simulink model "reglet_damping_variant_g"  (R2024b)
settings: Solver=VariableStepAuto  StartTime=0.0  StopTime=6  MaxStep=1e-3  RelTol=1e-3  AbsTol=1e-3  EnableMultiTasking=on
libraries: fl_lib x18, nesl_utility x6, simulink x1
CloseFcn:
  | try,close(h1_PermanentMagnetDCMotor),end
  | clear h1_PermanentMagnetDCMotor
  | 
  | clear simlog_PermanentMagnetDCMotor
Description:
  | Permanent Magnet DC Motor
settings Model: Creator=The MathWorks, Inc.  LastModifiedBy=thurard609
settings SolverCC: AutoScaleAbsTol=off  AlgebraicLoopSolver=TrustRegion
settings DataIOCC: LimitDataPoints=on  SaveFormat=Array  ReturnWorkspaceOutputs=off
settings OptimizationCC: ReuseModelBlockBuffer=off  LifeSpan=inf
settings DebuggingCC: SolverPrmCheckMsg=warning  UnconnectedInputMsg=warning  UnconnectedOutputMsg=warning  UnconnectedLineMsg=warning  AllowSymbolicDim=off  PregeneratedLibrarySubsystemCodeDiagnostic=none  SFUnexpectedBacktrackingDiag=warning  SFNoUnconditionalDefaultTransitionDiag=warning  SFExecutionAtInitializationDiag=none  ArithmeticOperatorsInVariantConditions=warning
settings HardwareCC: ProdBitPerPointer=32  ProdBitPerSizeT=32  ProdBitPerPtrDiffT=32  ProdLargestAtomicFloat=None  ProdIntDivRoundTo=Undefined  ProdEndianess=Unspecified  ProdWordSize=32  ProdHWDeviceType=32-bit Generic
settings ModelReferenceCC: EnableRefExpFcnMdlSchedulingChecks=on  PropagateSignalLabelsOutOfModel=off
settings SFSimCC: SimUseLocalCustomCode=off  CustomCodeUndefinedFunction=UseInterfaceOnly
settings RTWCC: RTWUseLocalCustomCode=off  GPUComputeCapability=3.5  DLArmComputeVersion=19.05
settings CodeAppCC: StateflowObjectComments=on
settings GRTTargetCC: TargetLangStandard=C89/C90 (ANSI)
settings ConfigComp: CovMetricSettings=dw  CovSaveCumulativeToWorkspaceVar=on  CovSaveSingleToWorkspaceVar=on  CovExternalEMLEnable=off  CovSFcnEnable=off
settings SimscapeCC: SimscapeLogType=all  SimscapeLogSimulationStatistics=on  SimscapeLogName=simlog_PermanentMagnetDCMotor  SimscapeLogDataHistory=10000

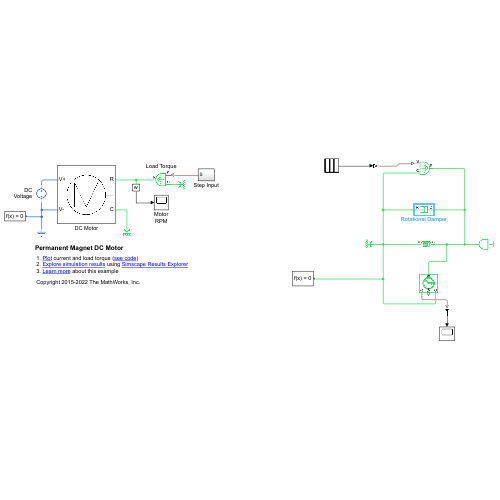
[thumbnail: Simulink's stored preview of the top-level diagram]
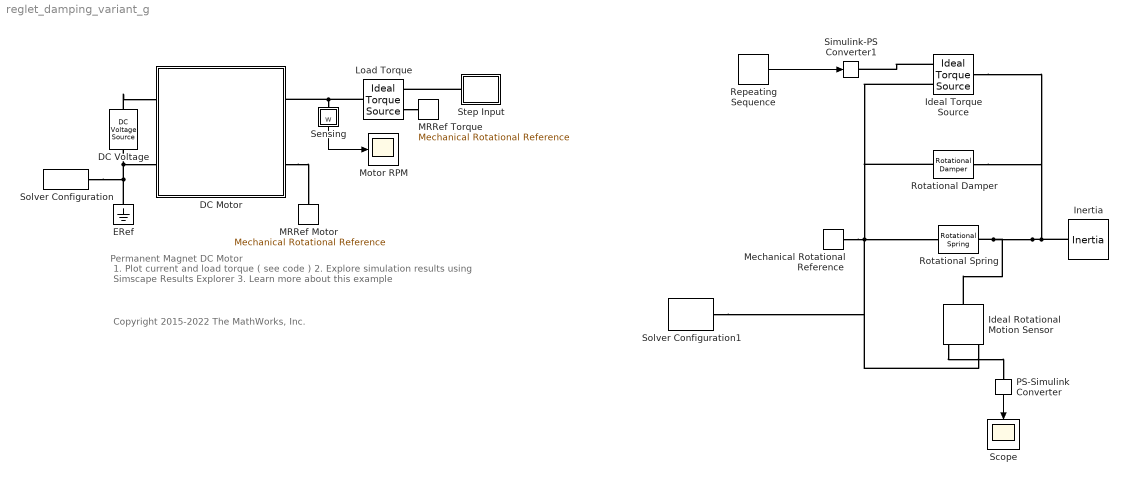
== system reglet_damping_variant_g ==
  note: 1. Plot current and load torque ( see code )
      | 2. Explore simulation results using Simscape Results Explorer
      | 3. Learn more about this example
  note: Permanent Magnet DC Motor
  note: Copyright 2015-2022 The MathWorks, Inc.
  DC Voltage : fl_lib/Electrical/Electrical Sources/DC Voltage Source  v0=1.5 V
  DC Motor : Subsystem  Tag=PublishSubsystem
      mask Display:
      | % Circle, in/out, and 'M'
      | image('PermanentMagnetDCMotorMaskIcon.png');
      | 
      | % % Circle
      | % plot(sin(0:0.1:2.2*pi)*0.9,cos(0:0.1:2.2*pi)*0.9);
      | %
      | % % In/out
      | % plot([-1.3 -0.9],[0 0]);
      | % plot([1.3 0.9],[0 0]);
      | %
      | % % 'M'
      | % plot([0.5 0.5],[-0.5 0.5]);
      | % plot([-0.5 -0.5],[-0.5 0.5]);
      | % plot([0.5 0],[0.5 -0.5]);
      | % plot([-0.5 0],[0.5 -0.5]);
      | 
      | % Plot points to set plot range
      | color('white');plot(1.5,1.5);plot(-1.5,-1.5)
      | color('black');
      | 
      | port_label('RConn',1,'R');
      | port_label('RConn',2,'C');
      | port_label('LConn',1,'V+');
      | port_label('LConn',2,'V-');
  ERef : fl_lib/Electrical/Electrical Elements/Electrical Reference
  Ideal Rotational Motion Sensor : fl_lib/Mechanical/Mechanical Sensors/Ideal Rotational Motion Sensor  reference=foundation.enum.MeasurementReference.difference  acceleration_port=false  velocity_port=true  position_port=true  wrap_angle=false  offset=0 rad
  Ideal Torque Source : fl_lib/Mechanical/Mechanical Sources/Ideal Torque Source
  Inertia : fl_lib/Mechanical/Rotational Elements/Inertia  inertia=9e-4 kg*m^2  num_ports=foundation.enum.numPorts2.one  w_specify=off  w_priority=High  w=0 rad/s  w_nominal_specify=off  w_nominal_value=1  w_nominal_unit=rad/s  t_specify=off  t_priority=None  t=0 N*m  t_nominal_specify=off  t_nominal_value=1  t_nominal_unit=N*m
  Load Torque : fl_lib/Mechanical/Mechanical Sources/Ideal Torque Source
  MRRef Motor : fl_lib/Mechanical/Rotational Elements/Mechanical Rotational Reference
  MRRef Torque : fl_lib/Mechanical/Rotational Elements/Mechanical Rotational Reference
  Mechanical Rotational Reference : fl_lib/Mechanical/Rotational Elements/Mechanical Rotational Reference
  Motor RPM : Scope
  PS-Simulink Converter : nesl_utility/PS-Simulink Converter  PhysicalDomain=network_engine_domain  SubClassName=ps_output  LeftPortType=input  RightPortType=output  PseudoPeriodic=off  Frequencies=[]  VectorFormat=inherit  Unit=rad  AffineConversion=off
  Repeating Sequence : simulink/Sources/Repeating Sequence  rep_seq_t=[0 0.01 0.02 0.03 6]  rep_seq_y=[0 0.05 0.05 0 0]
  Rotational Damper : fl_lib/Mechanical/Rotational Elements/Rotational Damper  D=1.661e-3 N*m*s/rad  w_specify=off  w_priority=None  w=0 rad/s  w_nominal_specify=off  w_nominal_value=1  w_nominal_unit=rad/s  t_specify=off  t_priority=None  t=0 N*m  t_nominal_specify=off  t_nominal_value=1  t_nominal_unit=N*m
  Rotational Spring : fl_lib/Mechanical/Rotational Elements/Rotational Spring  spr_rate=0.4476 N*m/rad  w_specify=off  w_priority=None  w=0 rad/s  w_nominal_specify=off  w_nominal_value=1  w_nominal_unit=rad/s  t_specify=off  t_priority=None  t=0 N*m  t_nominal_specify=off  t_nominal_value=1  t_nominal_unit=N*m  phi_specify=off  phi_priority=High  phi=0 rad  phi_nominal_specify=off  phi_nominal_value=1  phi_nominal_unit=rad
  Scope : Scope
  Sensing : Subsystem
      mask Display: disp('w');
  Simulink-PS Converter1 : nesl_utility/Simulink-PS Converter  PhysicalDomain=network_engine_domain  SubClassName=ps_input  LeftPortType=input  RightPortType=output  PseudoPeriodic=off  Frequencies=[]  NoiseDistribution=none  NoiseParameters=[]  Unit=N*m  AffineConversion=off  FilteringAndDerivatives=provide  SimscapeFilterOrder=1  InputFilterTimeConstant=0.001  UdotUserProvided=0
  Solver Configuration : nesl_utility/Solver Configuration  PhysicalDomain=network_engine_domain  SubClassName=solver  LeftPortType=input  RightPortType=generic  Tones=[]  Harmonics=[]  SimulateNoise=off  Profile=off  UseLocalSampling=off  EnableSwitchedLinearOptims=on  FrequencyDomain=off  UseCCode=off  RelTol=0.001  AbsTol=1e-06  MinStep=1e-09  ToWorkspace=off  RevertToSquareIcSolve=off  NumHomotopyIterations=100  PhasorMode=off  PhasorModeNumHarmonics=1  ConsistencySolver=NEWTON_XTOL_AFTER_FTOL  IndexReductionMethod=DerivativeReplacement  DoDC=off  ResidualTolerance=1e-9  ConsistencyTolSource=GLOBAL  ConsistencyAbsTol=0.001  ConsistencyRelTol=0.001  ConsistencyTolFactor=0.001  UseLocalSolver=off  LocalSolverChoice=NE_BACKWARD_EULER_ADVANCER  ResolveIndetEquations=on  FunctionEvalNumThread=1  LocalSolverSampleTime=.001  DoFixedCost=off  MaxNonlinIter=3  MaxModeIter=2  ComputeImpulses=off  ImpulseIterations=2  LinearAlgebra=auto  LinearAlgebraNumThread=0  EquationFormulation=NE_TIME_EF  DelaysMemoryBudget=1024  AutomaticFiltering=on  FilteringTimeConstant=0.001  PartitionStorageMethod=AS_NEEDED  PartitionMemoryBudget=1024  PartitionMethod=FAST  MultibodyUseLocalSolver=off  MultibodyLocalSolverChoice=ODE1  MultibodyLocalSolverSampleTime=0.001
  Solver Configuration1 : nesl_utility/Solver Configuration  PhysicalDomain=network_engine_domain  SubClassName=solver  LeftPortType=input  RightPortType=generic  Tones=[]  Harmonics=[]  SimulateNoise=off  Profile=off  UseLocalSampling=off  EnableSwitchedLinearOptims=on  FrequencyDomain=off  UseCCode=off  RelTol=0.001  AbsTol=1e-06  MinStep=1e-09  ToWorkspace=off  RevertToSquareIcSolve=off  NumHomotopyIterations=100  PhasorMode=off  PhasorModeNumHarmonics=1  ConsistencySolver=NEWTON_XTOL_AFTER_FTOL  IndexReductionMethod=DerivativeReplacement  DoDC=off  ResidualTolerance=1e-09  ConsistencyTolSource=GLOBAL  ConsistencyAbsTol=0.001  ConsistencyRelTol=0.001  ConsistencyTolFactor=0.001  UseLocalSolver=off  LocalSolverChoice=NE_BACKWARD_EULER_ADVANCER  ResolveIndetEquations=on  FunctionEvalNumThread=1  LocalSolverSampleTime=0.001  DoFixedCost=off  MaxNonlinIter=3  MaxModeIter=2  ComputeImpulses=off  ImpulseIterations=2  LinearAlgebra=auto  LinearAlgebraNumThread=0  EquationFormulation=NE_TIME_EF  DelaysMemoryBudget=1024  AutomaticFiltering=on  FilteringTimeConstant=0.001  PartitionStorageMethod=AS_NEEDED  PartitionMemoryBudget=1024  PartitionMethod=ROBUST  MultibodyUseLocalSolver=off  MultibodyLocalSolverChoice=ODE1  MultibodyLocalSolverSampleTime=0.001
  Step Input : Subsystem
  wires:
  Sensing/1(w) -> Motor RPM/1
  Repeating Sequence/1 -> Simulink-PS Converter1/1
  PS-Simulink Converter/1 -> Scope/1
  connections:
  ERef/LConn1 -- Solver Configuration/RConn1 -- DC Voltage/RConn1 -- DC Motor/LConn2
  DC Motor/RConn2 -- MRRef Motor/LConn1
  Load Torque/LConn1 -- DC Motor/RConn1 -- Sensing/LConn1
  DC Voltage/LConn1 -- DC Motor/LConn1
  Load Torque/RConn2 -- MRRef Torque/LConn1
  Step Input/LConn1 -- Load Torque/RConn1
  Rotational Spring/RConn1 -- Inertia/LConn1 -- Rotational Damper/RConn1 -- Ideal Torque Source/LConn1 -- Ideal Rotational Motion Sensor/LConn1
  Mechanical Rotational Reference/LConn1 -- Ideal Rotational Motion Sensor/RConn1 -- Solver Configuration1/RConn1 -- Rotational Spring/LConn1 -- Rotational Damper/LConn1 -- Ideal Torque Source/RConn2
  Ideal Torque Source/RConn1 -- Simulink-PS Converter1/RConn1
  Ideal Rotational Motion Sensor/RConn3 -- PS-Simulink Converter/LConn1

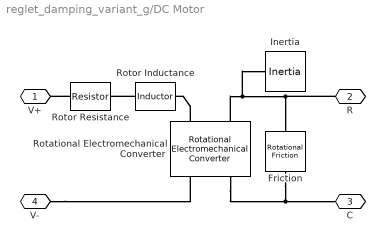
== system reglet_damping_variant_g/DC Motor ==
  Friction : fl_lib/Mechanical/Rotational Elements/Rotational Friction  brkwy_trq=0.02e-3 N*m  brkwy_vel=0.03347 rad/s  Col_trq=0.02e-3 N*m  visc_coef=0 N*m/(rad/s)  w_specify=off  w_priority=High  w=0 rad/s  w_nominal_specify=off  w_nominal_value=1  w_nominal_unit=rad/s  t_specify=off  t_priority=High  t=0 N*m  t_nominal_specify=off  t_nominal_value=1  t_nominal_unit=N*m
  Inertia : fl_lib/Mechanical/Rotational Elements/Inertia  inertia=0.01 g*cm^2  num_ports=foundation.enum.numPorts2.one  w_specify=off  w_priority=High  w=0 rad/s  w_nominal_specify=off  w_nominal_value=1  w_nominal_unit=rad/s  t_specify=off  t_priority=High  t=0 N*m  t_nominal_specify=off  t_nominal_value=1  t_nominal_unit=N*m
  Rotational Electromechanical Converter : fl_lib/Electrical/Electrical Elements/Rotational Electromechanical Converter  K=0.072e-3*60/(2*pi) s*V/rad  i_specify=off  i_priority=High  i=0 A  i_nominal_specify=off  i_nominal_value=1  i_nominal_unit=A  v_specify=off  v_priority=High  v=0 V  v_nominal_specify=off  v_nominal_value=1  v_nominal_unit=V  t_specify=off  t_priority=High  t=0 N*m  t_nominal_specify=off  t_nominal_value=1  t_nominal_unit=N*m  w_specify=off  w_priority=High  w=0 rad/s  w_nominal_specify=off  w_nominal_value=1  w_nominal_unit=rad/s
  Rotor Inductance : fl_lib/Electrical/Electrical Elements/Inductor  l=12e-6 H  r=0 Ohm  g=1e-09 1/Ohm  i_specify=off  i_priority=High  i=0 A  i_nominal_specify=off  i_nominal_value=1  i_nominal_unit=A  v_specify=off  v_priority=High  v=0 V  v_nominal_specify=off  v_nominal_value=1  v_nominal_unit=V  i_L_specify=on  i_L_priority=High  i_L=0 A  i_L_nominal_specify=off  i_L_nominal_value=1  i_L_nominal_unit=A
  Rotor Resistance : fl_lib/Electrical/Electrical Elements/Resistor  Tag=Factory Generic  R=3.9 Ohm  i_specify=off  i_priority=High  i=0 A  i_nominal_specify=off  i_nominal_value=1  i_nominal_unit=A  v_specify=off  v_priority=High  v=0 V  v_nominal_specify=off  v_nominal_value=1  v_nominal_unit=V
  V+ : PMIOPort  Side=Left
  R : PMIOPort  Port=2  Side=Right
  C : PMIOPort  Port=3  Side=Right
  V- : PMIOPort  Port=4  Side=Left
  connections:
  Rotational Electromechanical Converter/LConn1 -- Rotor Inductance/RConn1
  V-/RConn1 -- Rotational Electromechanical Converter/RConn1
  Rotor Resistance/LConn1 -- V+/RConn1
  Rotor Inductance/LConn1 -- Rotor Resistance/RConn1
  Rotational Electromechanical Converter/LConn2 -- R/RConn1 -- Friction/LConn1 -- Inertia/LConn1
  Rotational Electromechanical Converter/RConn2 -- C/RConn1 -- Friction/RConn1

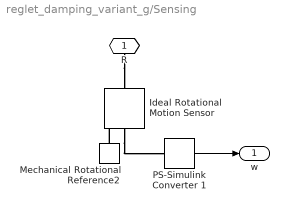
== system reglet_damping_variant_g/Sensing ==
  Ideal Rotational Motion Sensor : fl_lib/Mechanical/Mechanical Sensors/Ideal Rotational Motion Sensor  reference=foundation.enum.MeasurementReference.difference  acceleration_port=false  velocity_port=true  position_port=true  wrap_angle=simscape.enum.onoff.off  offset=0 rad
  Mechanical Rotational Reference2 : fl_lib/Mechanical/Rotational Elements/Mechanical Rotational Reference
  PS-Simulink Converter 1 : nesl_utility/PS-Simulink Converter  PhysicalDomain=network_engine_domain  SubClassName=ps_output  LeftPortType=input  RightPortType=output  PseudoPeriodic=off  Frequencies=[]  VectorFormat=1-D array  Unit=rpm  AffineConversion=off
  R : PMIOPort  Side=Left
  w : Outport  VectorParamsAs1DForOutWhenUnconnected=off
  wires:
  PS-Simulink Converter 1/1 -> w/1
  connections:
  Ideal Rotational Motion Sensor/RConn2 -- PS-Simulink Converter 1/LConn1
  Mechanical Rotational Reference2/LConn1 -- Ideal Rotational Motion Sensor/RConn1
  R/RConn1 -- Ideal Rotational Motion Sensor/LConn1

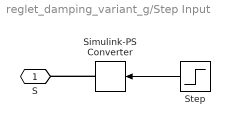
== system reglet_damping_variant_g/Step Input ==
  Simulink-PS Converter : nesl_utility/Simulink-PS Converter  PhysicalDomain=network_engine_domain  SubClassName=ps_input  LeftPortType=input  RightPortType=output  PseudoPeriodic=off  Frequencies=[]  NoiseDistribution=none  NoiseParameters=[]  Unit=1  AffineConversion=off  FilteringAndDerivatives=zero  SimscapeFilterOrder=1  InputFilterTimeConstant=.001  UdotUserProvided=0
  Step : Step  Time=0.1  After=-0.24e-3  SampleTime=0
  S : PMIOPort  Side=Left
  wires:
  Step/1 -> Simulink-PS Converter/1
  connections:
  Simulink-PS Converter/RConn1 -- S/RConn1
